simulink model "Controller_BoP"  (R2026a)
settings: Solver=FixedStepDiscrete  StopTime=10  FixedStep=Ts_ctrl
InitFcn:
  | init_Controller_BoP
undefined symbols (not defined in the file or in its folder): BoP_e_clip, BoP_Kd, BoP_Ki, BoP_Kp, BoP_Nq, BoP_th_lim, BoP_Ts, BoP_v_int, Ts_ctrl
Description:
  | Controlador Ball on Plate, un eje. Ley en bop_ley_control.m (Etapa C). Entradas r, x_hat, v_hat del Kalman y habilitado; salida th_cmd en rad. Referencia intocable: las variantes son copias con otro nombre.
settings Model: Creator=ablopez@estudiantes.ie.tec.ac.cr  LastModifiedBy=ablopez@estudiantes.ie.tec.ac.cr
settings HardwareCC: ProdHWDeviceType=Generic->32-bit Embedded Processor
settings RTWCC: SystemTargetFile=ert.tlc  GenCodeOnly=on  GenerateReport=on  PortableWordSizes=on  Description=Embedded Coder
settings ERTTargetCC: GenerateSampleERTMain=on  CodeInterfacePackaging=Reusable function

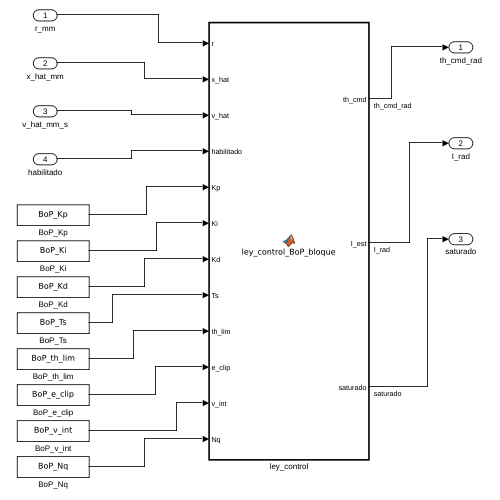
[thumbnail: Simulink's stored preview of the top-level diagram]
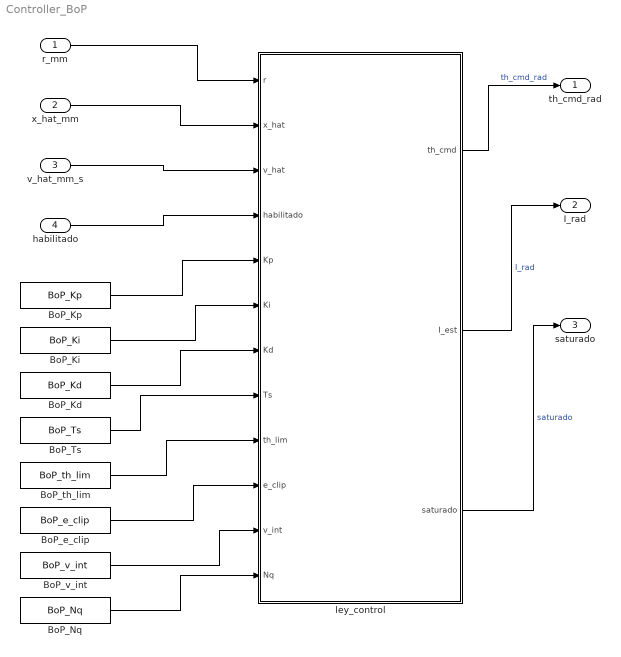
== system Controller_BoP ==
  r_mm : Inport  OutDataTypeStr=double  PortDimensions=1  SampleTime=Ts_ctrl  Interpolate=off
  x_hat_mm : Inport  Port=2  OutDataTypeStr=double  PortDimensions=1  SampleTime=Ts_ctrl  Interpolate=off
  v_hat_mm_s : Inport  Port=3  OutDataTypeStr=double  PortDimensions=1  SampleTime=Ts_ctrl  Interpolate=off
  habilitado : Inport  Port=4  OutDataTypeStr=boolean  PortDimensions=1  SampleTime=Ts_ctrl  Interpolate=off
  BoP_Kd : Constant  Value=BoP_Kd  OutDataTypeStr=double
  BoP_Ki : Constant  Value=BoP_Ki  OutDataTypeStr=double
  BoP_Kp : Constant  Value=BoP_Kp  OutDataTypeStr=double
  BoP_Nq : Constant  Value=BoP_Nq  OutDataTypeStr=double
  BoP_Ts : Constant  Value=BoP_Ts  OutDataTypeStr=double
  BoP_e_clip : Constant  Value=BoP_e_clip  OutDataTypeStr=double
  BoP_th_lim : Constant  Value=BoP_th_lim  OutDataTypeStr=double
  BoP_v_int : Constant  Value=BoP_v_int  OutDataTypeStr=double
  ley_control : MATLAB Function  TreatAsAtomicUnit=on
  th_cmd_rad : Outport
  I_rad : Outport  Port=2
  saturado : Outport  Port=3
  wires:
  r_mm/1 -> ley_control/1(r)
  x_hat_mm/1 -> ley_control/2(x_hat)
  v_hat_mm_s/1 -> ley_control/3(v_hat)
  habilitado/1 -> ley_control/4(habilitado)
  BoP_Kp/1 -> ley_control/5(Kp)
  BoP_Ki/1 -> ley_control/6(Ki)
  BoP_Kd/1 -> ley_control/7(Kd)
  BoP_Ts/1 -> ley_control/8(Ts)
  BoP_th_lim/1 -> ley_control/9(th_lim)
  BoP_e_clip/1 -> ley_control/10(e_clip)
  BoP_v_int/1 -> ley_control/11(v_int)
  BoP_Nq/1 -> ley_control/12(Nq)
  ley_control/1(th_cmd) -> th_cmd_rad/1  "th_cmd_rad"
  ley_control/2(I_est) -> I_rad/1  "I_rad"
  ley_control/3(saturado) -> saturado/1  "saturado"

== matlab function Controller_BoP/ley_control ==
  data: r input; th_cmd output; x_hat input; v_hat input; habilitado input; Kp input; Ki input; Kd input; Ts input; th_lim input; e_clip input; v_int input; Nq input; I_est output; saturado output
function [th_cmd, I_est, saturado] = ley_control_BoP_bloque(r, x_hat, v_hat, habilitado, ...
    Kp, Ki, Kd, Ts, th_lim, e_clip, v_int, Nq)
%LEY_CONTROL_BOP_BLOQUE Funcion principal del bloque MATLAB Function de Controller_BoP.slx.
%
% E0_build_Controller_BoP copia este archivo, seguido de bop_ley_control.m,
% dentro del bloque "ley_control". El modelo queda autocontenido: no depende
% de archivos externos despues de construido.
%
% Un eje. Se llama una vez por cuadro de camara (Ts).
%   r [mm], x_hat [mm], v_hat [mm/s]   referencia y estado del Kalman
%   habilitado (logico)                false: plato horizontal (th_cmd = 0) y
%                                      estado interno en cero (arranque, sin
%                                      bola, perdida de comunicacion)
%   Kp ... Nq                          parametros calibrables (init_Controller_BoP)
%   th_cmd [rad]                       inclinacion pedida al plato
%   I_est [rad]                        integrador (para registro y verificacion)
%   saturado (logico)                  th_cmd saturado en este paso
% Estado interno (persistente): I [rad], nq [cuadros con la bola quieta].
%#codegen

persistent I nq
if isempty(I)
    I = 0;
    nq = 0;
end
if habilitado
    [th_cmd, I, nq, ~, saturado, ~] = bop_ley_control(x_hat, v_hat, r, I, nq, ...
        Kp, Ki, Kd, Ts, th_lim, e_clip, v_int, Nq, true, true);
else
    th_cmd = 0;
    I = 0;
    nq = 0;
    saturado = false;
end
I_est = I;
end


function [th_cmd, I_n, nq_n, u, saturado, integra] = bop_ley_control(x_hat, v_hat, r, I, nq, ...
    Kp, Ki, Kd, Ts, th_lim, e_clip, v_int, Nq, usar_aw, saturar)
%BOP_LEY_CONTROL Ley de control de UN eje, un paso (escalares, apta para codigo).
%
%   [th_cmd, I_n, nq_n, u, saturado, integra] = bop_ley_control(x_hat, v_hat, r, I, nq, ...
%       Kp, Ki, Kd, Ts, th_lim, e_clip, v_int, Nq, usar_aw, saturar)
%
% UNICA FUENTE del algoritmo. La usan:
%   - el MIL (etapaD, a traves de bop_controlador_paso), y
%   - el bloque MATLAB Function de Controller_BoP.slx (etapaE): el script
%     E0_build_Controller_BoP copia este archivo dentro del bloque.
% Si se cambia aqui, hay que reconstruir el modelo y repetir E1 (equivalencia).
%
% Entradas:  x_hat [mm], v_hat [mm/s], r [mm], I [rad], nq [cuadros]
% Parametros: Kp [rad/mm], Ki [rad/(mm s)], Kd [rad/(mm/s)], Ts [s],
%             th_lim [rad], e_clip [mm], v_int [mm/s], Nq [cuadros]
%             usar_aw, saturar: logicos (en el modelo del controlador, true)
% Salidas:   th_cmd [rad], I_n y nq_n (estado del paso siguiente),
%            u [rad] (sin saturar), saturado, integra (logicos)
%
% Ley (eps = x_hat - r, ganancias positivas: th > 0 acelera la bola hacia -x):
%   u      = Kp*eps + I + Kd*v_hat
%   th_cmd = sat(u, +-th_lim)
%   nq_n   = nq + 1 si |v_hat| < v_int, si no 0
%   I_n    = I + Ki*Ts*sat(eps, +-e_clip)  si nq_n >= max(Nq,1) y no
%            (usar_aw y saturado y sign(eps) == sign(u));  si no, I_n = I
%#codegen

eps_ = x_hat - r;
u = Kp*eps_ + I + Kd*v_hat;
if saturar
    th_cmd = min(max(u, -th_lim), th_lim);
else
    th_cmd = u;
end
saturado = (th_cmd ~= u);
congelar = usar_aw && saturado && (sign(eps_) == sign(u));

if abs(v_hat) < v_int
    nq_n = nq + 1;
else
    nq_n = 0;
end
integra = ~congelar && (nq_n >= max(Nq, 1));
if integra
    I_n = I + Ki*Ts*min(max(eps_, -e_clip), e_clip);
else
    I_n = I;
end
end
